simulink model "untitled"  (R2021b)
settings: Solver=VariableStepAuto  StartTime=0.0  StopTime=50  RelTol=1e-3
settings Model: Creator=kourosh  LastModifiedBy=kourosh

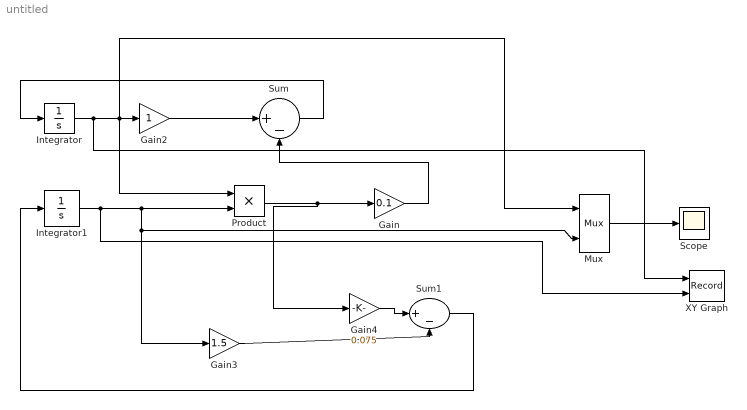
== system untitled ==
  Gain : Gain  Gain=0.1
  Gain2 : Gain
  Gain3 : Gain  Gain=1.5
  Gain4 : Gain  Gain=0.075
  Integrator : Integrator  InitialCondition=10  ContinuousStateAttributes="\"x\""
  Integrator1 : Integrator  InitialCondition=5
  Mux : Mux  Inputs=2
  Product : Product
  Scope : Scope
  Sum : Sum  Inputs=|+-
  Sum1 : Sum  Inputs=|+-
  XY Graph : Record  FileSettingsInternal="{\"entries\":[{\"content\":{\"excelSettings\":{\"content\":{},\"type\":\"Streamout.ExcelSettings\"}},\"type\":\"Streamout.FileSettingStorage\",\"uuid\":\"149b6535-eb6b-4e87-ba3b-7c4b531b1a96\"}],\"packageUris\":[\"http://schema.mathworks.com/mf0/streamout_blocks/R2020a\"],\"version\":\"1.0\"}"  Layout=[1 1]  SignalsInternal="{\"entries\":[{\"content\":{\"signals\":[{\"content\":{\"blockPath\":[\"untitled/XY Graph\"],\"channel\":[],\"dimensions\":[1],\"domain\":\"untitled/XY Graph\",\"lineColor\":\"#a2142f\",\"plots\":[1],\"port\":1,\"sid\":[\"\"],\"signalID\":236,\"signalName\":\"Integrator\"},\"type\":\"RecordBlkView.Signal\",\"uuid\":\"9ad0677c-6ce4-4e61-995c-2a9ecc5802ef\"},{\"content\":{\"blockPath\":[\"untitled/XY Graph\"],\"channel\":[],\"dimensions\":[1],\"domain\":\"untitled/XY Graph\",\"lineColor\":\"#139fff\",\"plots\":[1],\"port\":2,\"sid\":[\"\"],\"signalID\":240,\"signalName\":\"Integrator1\"},\"type\":\"RecordBlkView.Signal\",\"uuid\":\"ba98dca9-917c-4d95-adf7-4219e2050686\"}]},\"type\":\"RecordBlkView.InputSignals\",\"uuid\":\"c9e6c419-992c-407f-bac9-e0d050ff6187\"}],\"packageUris\":[\"http://schema.mathworks.com/mf0/streamout_blocks/R2020a\"],\"version\":\"1.0\"}"  VisualizationBindings="{\"xyplotplugin\":{\"info\":[{\"series\":[{\"bindingParametersList\":[{\"parameter\":\"X-Axis\",\"signalID\":236,\"signalName\":\"Integrator\"},{\"parameter\":\"Y-Axis\",\"signalID\":240,\"signalName\":\"Integrator1\"}],\"seriesID\":44328}],\"subplotID\":1}]}}"  CompatibilityTag=XY
  wires:
  Integrator/1 -> XY Graph/1, Product/1, Mux/1, Gain2/1
  Integrator1/1 -> XY Graph/2, Gain3/1, Mux/2, Product/2
  Gain2/1 -> Sum/1
  Product/1 -> Gain4/1, Gain/1
  Gain/1 -> Sum/2
  Sum/1 -> Integrator/1
  Gain3/1 -> Sum1/2
  Sum1/1 -> Integrator1/1
  Mux/1 -> Scope/1
  Gain4/1 -> Sum1/1
